simulink library "QB_pacer_lib_2024b"  (R2024b)
settings: Solver=ode45  StartTime=0.0  StopTime=10.0  RelTol=1e-3  EnableMultiTasking=on
settings Model: Creator=gvallabh  LastModifiedBy=cpetrocelli
settings SolverCC: AlgebraicLoopSolver=TrustRegion
settings DataIOCC: LimitDataPoints=on  SaveFormat=Array  SignalLoggingSaveFormat=ModelDataLogs  ReturnWorkspaceOutputs=off
settings OptimizationCC: ReuseModelBlockBuffer=off  ExpressionDepthLimit=2147483647  LifeSpan=inf
settings DebuggingCC: UnderspecifiedInitializationDetection=Classic  MergeDetectMultiDrivingBlocksExec=none  SolverPrmCheckMsg=warning  FcnCallInpInsideContextMsg=warning  UnconnectedInputMsg=warning  UnconnectedOutputMsg=warning  UnconnectedLineMsg=warning  StateNameClashWarn=warning  SFUnexpectedBacktrackingDiag=warning  SFNoUnconditionalDefaultTransitionDiag=warning  SFExecutionAtInitializationDiag=none  ArithmeticOperatorsInVariantConditions=warning
settings HardwareCC: ProdBitPerPointer=32  ProdBitPerSizeT=32  ProdBitPerPtrDiffT=32  ProdLargestAtomicFloat=None  ProdIntDivRoundTo=Undefined  ProdEndianess=Unspecified  ProdWordSize=32  ProdHWDeviceType=32-bit Generic
settings ModelReferenceCC: EnableRefExpFcnMdlSchedulingChecks=on  PropagateSignalLabelsOutOfModel=off
settings SFSimCC: SimUseLocalCustomCode=off  CustomCodeUndefinedFunction=UseInterfaceOnly
settings RTWCC: RTWUseLocalCustomCode=off  GPUComputeCapability=3.5  DLArmComputeVersion=19.05
settings CodeAppCC: StateflowObjectComments=on
settings GRTTargetCC: TargetLangStandard=C89/C90 (ANSI)  CombineOutputUpdateFcns=off  GRTInterface=on
settings ConfigComp: CovMetricSettings=dw  CovSaveCumulativeToWorkspaceVar=on  CovSaveSingleToWorkspaceVar=on  CovExternalEMLEnable=off  CovSFcnEnable=off

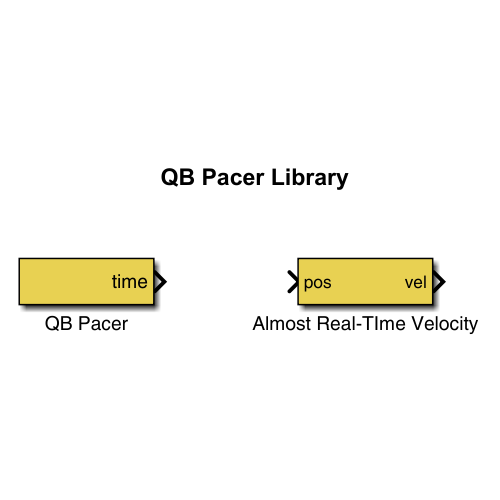
[thumbnail: Simulink's stored preview of the top-level diagram]
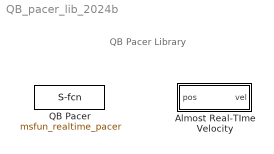
== system QB_pacer_lib_2024b ==
  note: QB Pacer Library
  Almost Real-TIme Velocity : Subsystem  mask(Almost Real-Time Velocity){}
      mask help:
      | Uses Real-Time Pacer to compute an almost real-time velocity.
      |
      | POS = position to use as reference
      | VEL = velocity (pos unit/second)
  QB Pacer : M-S-Function  AncestorBlock=realtime_pacer_lib/Real-Time Pacer  FunctionName=msfun_realtime_pacer  Parameters=simTimePerRealTime  mask(RealTime_Pacer){simTimePerRealTime=1}
      mask prompts: simTimePerRealTime "Speedup (Simulation Time / Real Time):"
      mask help:
      | Slow down a simulation to track real (i.e., wall clock) elapsed time.
      |
      | "Speedup" specifies the ratio between simulation time and real time
      |  Speedup = N => N sec. of simulation time per sec. of real time
      |  Speedup can be fractional (e.g., 0.5, 1.3).
      |  Speedup = inf => allow simulation to run at full speed
      |
      | Click on the Help button for details.
      settings: LibrarySourceBlock=realtime_pacer_lib/Real-Time Pacer
      mask Help: web('realtime_pacer_help.html', '-helpbrowser')
      mask Display:
      | %fprintf('QB Pacer\nSpeedup = %g', simTimePerRealTime)
      | port_label('output',1,'time');

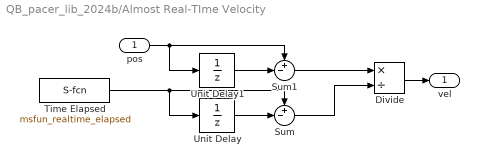
== system QB_pacer_lib_2024b/Almost Real-TIme Velocity ==
  pos : Inport
  Divide : Product  Inputs=*/
  Sum : Sum  Inputs=+-|
  Sum1 : Sum  Inputs=+-|
  Time Elapsed : M-S-Function  AncestorBlock=realtime_pacer_lib/Real-Time Pacer  FunctionName=msfun_realtime_elapsed  mask(Time Elapsed){}
      settings: LibrarySourceBlock=realtime_pacer_lib/Real-Time Pacer
      mask Display: port_label('output',1,'time');
  Unit Delay : UnitDelay  SampleTime=-1  HasFrameUpgradeWarning=on
  Unit Delay1 : UnitDelay  SampleTime=-1  HasFrameUpgradeWarning=on
  vel : Outport  VectorParamsAs1DForOutWhenUnconnected=off
  wires:
  Time Elapsed/1 -> Sum/1, Unit Delay/1
  Divide/1 -> vel/1
  Sum/1 -> Divide/2
  Sum1/1 -> Divide/1
  Unit Delay1/1 -> Sum1/2
  pos/1 -> Unit Delay1/1, Sum1/1
  Unit Delay/1 -> Sum/2
